simulink model "model_file_sim1"  (R2026b)
settings: Solver=FixedStepAuto  StopTime=stopTimeSimu  FixedStep=Ts
values from neighbouring files (symbols this model uses):
  Rc_alu = 11.0    (= 11)    [model.m]
  Rc_fan = 3.33    [model.m]
  Rc_fan1 = 3.33    [model.m]
  Rc_pet = 28.9    [model.m]
  Rc_pet1 = 28.9    [model.m]
  Rth_alu = 1.84 / 2    (= 0.92)    [model.m]
  Rth_alu2 = 1.84 / 2    (= 0.92)    [model.m]
  Rth_fan = 65.0 / 2    (= 32.5)    [model.m]
  Rth_fan2 = 65.0 / 2    (= 32.5)    [model.m]
  Rth_pet = 22.5 / 2    (= 11.25)    [model.m]
  Rth_pet2 = 22.5 / 2    (= 11.25)    [model.m]
  Rth_sen = 180.0    (= 180)    [model.m]
  Rv = 3.1    [model.m]
  Ts = 1    [R_from_logs.mat]    (also in estimate_R.m; kalman_manuel.m; kalman_simulink.m; model_file.m)
libraries: fl_lib x27, nesl_utility x4
settings Model: Creator=33683  LastModifiedBy=nael
settings DataIOCC: DSMLogging=off  ExternalInput=data_in  LoadExternalInput=on  ReturnWorkspaceOutputs=off  SaveOutput=off  SaveTime=off  SignalLogging=off
settings RTWCC: GPUComputeCapability=5.0
settings SimscapeCC: SimscapeUseEnergyAccounting=off

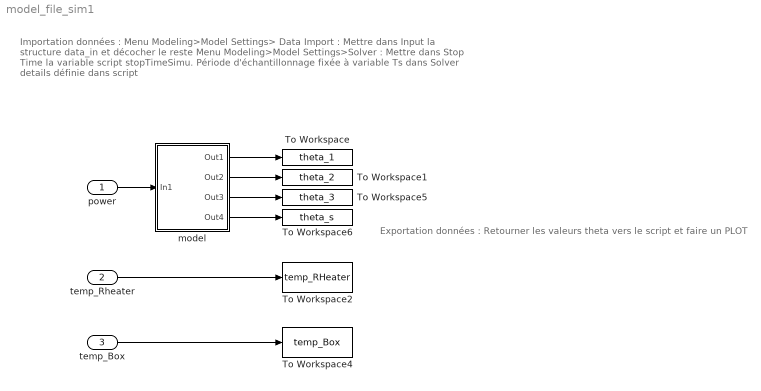
== system model_file_sim1 ==
  note: Importation données :
      | Menu Modeling>Model Settings> Data Import : Mettre dans Input la structure data_in et décocher le reste
      | Menu Modeling>Model Settings>Solver : Mettre dans Stop Time la variable script stopTimeSimu. Période d'échantillonnage fixée à variable Ts dans Solver details définie dans script
  note: Exportation données : Retourner les valeurs theta vers le script et faire un PLOT
  power : Inport
  temp_Rheater : Inport  Port=2
  temp_Box : Inport  Port=3
  To Workspace : ToWorkspace  VariableName=theta_1  SampleTime=Ts
  To Workspace1 : ToWorkspace  VariableName=theta_2  SampleTime=Ts
  To Workspace2 : ToWorkspace  VariableName=temp_RHeater  SampleTime=Ts
  To Workspace4 : ToWorkspace  VariableName=temp_Box  SampleTime=Ts
  To Workspace5 : ToWorkspace  VariableName=theta_3  SampleTime=Ts
  To Workspace6 : ToWorkspace  VariableName=theta_s  SampleTime=Ts
  model : Subsystem
  wires:
  temp_Rheater/1 -> To Workspace2/1
  temp_Box/1 -> To Workspace4/1
  power/1 -> model/1(In1)
  model/1(Out1) -> To Workspace/1
  model/2(Out2) -> To Workspace1/1
  model/3(Out3) -> To Workspace5/1
  model/4(Out4) -> To Workspace6/1

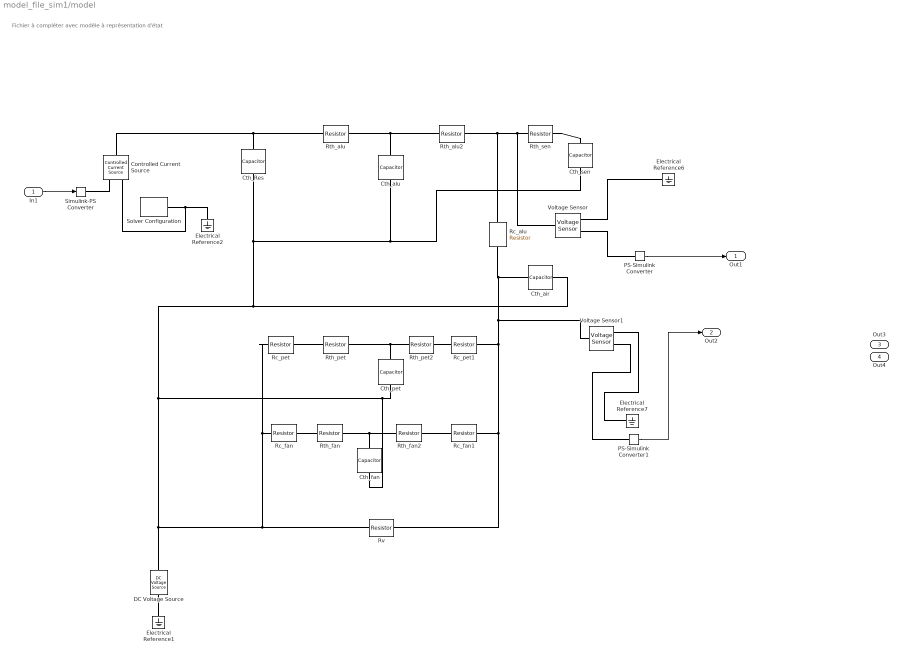
== system model_file_sim1/model ==
  note: Fichier à compléter avec modèle à représentation d'état
  In1 : Inport
  Controlled Current Source : fl_lib/Electrical/Electrical Sources/Controlled Current Source
  Cth_Res : fl_lib/Electrical/Electrical Elements/Capacitor  c=Cth_Res F  r=0 Ohm  g=0 1/Ohm  i_specify=off  i_priority=None  i=0 A  i_nominal_specify=off  i_nominal_value=1  i_nominal_unit=A  v_specify=off  v_priority=None  v=0 V  v_nominal_specify=off  v_nominal_value=1  v_nominal_unit=V  vc_specify=off  vc_priority=High  vc=0 V  vc_nominal_specify=off  vc_nominal_value=1  vc_nominal_unit=V
  Cth_air : fl_lib/Electrical/Electrical Elements/Capacitor  c=Cth_air F  r=0 Ohm  g=0 1/Ohm  i_specify=off  i_priority=None  i=0 A  i_nominal_specify=off  i_nominal_value=1  i_nominal_unit=A  v_specify=off  v_priority=None  v=0 V  v_nominal_specify=off  v_nominal_value=1  v_nominal_unit=V  vc_specify=off  vc_priority=High  vc=0 V  vc_nominal_specify=off  vc_nominal_value=1  vc_nominal_unit=V
  Cth_alu : fl_lib/Electrical/Electrical Elements/Capacitor  c=Cth_alu F  r=0 Ohm  g=0 1/Ohm  i_specify=off  i_priority=None  i=0 A  i_nominal_specify=off  i_nominal_value=1  i_nominal_unit=A  v_specify=off  v_priority=None  v=0 V  v_nominal_specify=off  v_nominal_value=1  v_nominal_unit=V  vc_specify=off  vc_priority=High  vc=0 V  vc_nominal_specify=off  vc_nominal_value=1  vc_nominal_unit=V
  Cth_fan : fl_lib/Electrical/Electrical Elements/Capacitor  c=Cth_fan F  r=0 Ohm  g=0 1/Ohm  i_specify=off  i_priority=None  i=0 A  i_nominal_specify=off  i_nominal_value=1  i_nominal_unit=A  v_specify=off  v_priority=None  v=0 V  v_nominal_specify=off  v_nominal_value=1  v_nominal_unit=V  vc_specify=off  vc_priority=High  vc=0 V  vc_nominal_specify=off  vc_nominal_value=1  vc_nominal_unit=V
  Cth_pet : fl_lib/Electrical/Electrical Elements/Capacitor  c=Cth_pet F  r=0 Ohm  g=0 1/Ohm  i_specify=off  i_priority=None  i=0 A  i_nominal_specify=off  i_nominal_value=1  i_nominal_unit=A  v_specify=off  v_priority=None  v=0 V  v_nominal_specify=off  v_nominal_value=1  v_nominal_unit=V  vc_specify=off  vc_priority=High  vc=0 V  vc_nominal_specify=off  vc_nominal_value=1  vc_nominal_unit=V
  Cth_sen : fl_lib/Electrical/Electrical Elements/Capacitor  c=Cth_sen F  r=0 Ohm  g=0 1/Ohm  i_specify=off  i_priority=None  i=0 A  i_nominal_specify=off  i_nominal_value=1  i_nominal_unit=A  v_specify=off  v_priority=None  v=0 V  v_nominal_specify=off  v_nominal_value=1  v_nominal_unit=V  vc_specify=off  vc_priority=High  vc=0 V  vc_nominal_specify=off  vc_nominal_value=1  vc_nominal_unit=V
  DC Voltage Source : fl_lib/Electrical/Electrical Sources/DC Voltage Source  v0=22 V
  Electrical Reference{1..2,6..7} (4 alike) : fl_lib/Electrical/Electrical Elements/Electrical Reference
  PS-Simulink Converter : nesl_utility/PS-Simulink Converter  PhysicalDomain=network_engine_domain  SubClassName=ps_output  LeftPortType=input  RightPortType=output  PseudoPeriodic=off  Frequencies=[]  VectorFormat=inherit  Unit=inherit  AffineConversion=off
  PS-Simulink Converter1 : nesl_utility/PS-Simulink Converter  PhysicalDomain=network_engine_domain  SubClassName=ps_output  LeftPortType=input  RightPortType=output  PseudoPeriodic=off  Frequencies=[]  VectorFormat=inherit  Unit=inherit  AffineConversion=off
  Rc_alu : fl_lib/Electrical/Electrical Elements/Resistor  R=Rc_alu Ohm  i_specify=off  i_priority=None  i=0 A  i_nominal_specify=off  i_nominal_value=1  i_nominal_unit=A  v_specify=off  v_priority=None  v=0 V  v_nominal_specify=off  v_nominal_value=1  v_nominal_unit=V
  Rc_fan : fl_lib/Electrical/Electrical Elements/Resistor  R=Rc_fan Ohm  i_specify=off  i_priority=None  i=0 A  i_nominal_specify=off  i_nominal_value=1  i_nominal_unit=A  v_specify=off  v_priority=None  v=0 V  v_nominal_specify=off  v_nominal_value=1  v_nominal_unit=V
  Rc_fan1 : fl_lib/Electrical/Electrical Elements/Resistor  R=Rc_fan1 Ohm  i_specify=off  i_priority=None  i=0 A  i_nominal_specify=off  i_nominal_value=1  i_nominal_unit=A  v_specify=off  v_priority=None  v=0 V  v_nominal_specify=off  v_nominal_value=1  v_nominal_unit=V
  Rc_pet : fl_lib/Electrical/Electrical Elements/Resistor  R=Rc_pet Ohm  i_specify=off  i_priority=None  i=0 A  i_nominal_specify=off  i_nominal_value=1  i_nominal_unit=A  v_specify=off  v_priority=None  v=0 V  v_nominal_specify=off  v_nominal_value=1  v_nominal_unit=V
  Rc_pet1 : fl_lib/Electrical/Electrical Elements/Resistor  R=Rc_pet1 Ohm  i_specify=off  i_priority=None  i=0 A  i_nominal_specify=off  i_nominal_value=1  i_nominal_unit=A  v_specify=off  v_priority=None  v=0 V  v_nominal_specify=off  v_nominal_value=1  v_nominal_unit=V
  Rth_alu : fl_lib/Electrical/Electrical Elements/Resistor  R=Rth_alu Ohm  i_specify=off  i_priority=None  i=0 A  i_nominal_specify=off  i_nominal_value=1  i_nominal_unit=A  v_specify=off  v_priority=None  v=0 V  v_nominal_specify=off  v_nominal_value=1  v_nominal_unit=V
  Rth_alu2 : fl_lib/Electrical/Electrical Elements/Resistor  R=Rth_alu2 Ohm  i_specify=off  i_priority=None  i=0 A  i_nominal_specify=off  i_nominal_value=1  i_nominal_unit=A  v_specify=off  v_priority=None  v=0 V  v_nominal_specify=off  v_nominal_value=1  v_nominal_unit=V
  Rth_fan : fl_lib/Electrical/Electrical Elements/Resistor  R=Rth_fan Ohm  i_specify=off  i_priority=None  i=0 A  i_nominal_specify=off  i_nominal_value=1  i_nominal_unit=A  v_specify=off  v_priority=None  v=0 V  v_nominal_specify=off  v_nominal_value=1  v_nominal_unit=V
  Rth_fan2 : fl_lib/Electrical/Electrical Elements/Resistor  R=Rth_fan2 Ohm  i_specify=off  i_priority=None  i=0 A  i_nominal_specify=off  i_nominal_value=1  i_nominal_unit=A  v_specify=off  v_priority=None  v=0 V  v_nominal_specify=off  v_nominal_value=1  v_nominal_unit=V
  Rth_pet : fl_lib/Electrical/Electrical Elements/Resistor  R=Rth_pet Ohm  i_specify=off  i_priority=None  i=0 A  i_nominal_specify=off  i_nominal_value=1  i_nominal_unit=A  v_specify=off  v_priority=None  v=0 V  v_nominal_specify=off  v_nominal_value=1  v_nominal_unit=V
  Rth_pet2 : fl_lib/Electrical/Electrical Elements/Resistor  R=Rth_pet2 Ohm  i_specify=off  i_priority=None  i=0 A  i_nominal_specify=off  i_nominal_value=1  i_nominal_unit=A  v_specify=off  v_priority=None  v=0 V  v_nominal_specify=off  v_nominal_value=1  v_nominal_unit=V
  Rth_sen : fl_lib/Electrical/Electrical Elements/Resistor  R=Rth_sen Ohm  i_specify=off  i_priority=None  i=0 A  i_nominal_specify=off  i_nominal_value=1  i_nominal_unit=A  v_specify=off  v_priority=None  v=0 V  v_nominal_specify=off  v_nominal_value=1  v_nominal_unit=V
  Rv : fl_lib/Electrical/Electrical Elements/Resistor  R=Rv Ohm  i_specify=off  i_priority=None  i=0 A  i_nominal_specify=off  i_nominal_value=1  i_nominal_unit=A  v_specify=off  v_priority=None  v=0 V  v_nominal_specify=off  v_nominal_value=1  v_nominal_unit=V
  Simulink-PS Converter : nesl_utility/Simulink-PS Converter  PhysicalDomain=network_engine_domain  SubClassName=ps_input  LeftPortType=input  RightPortType=output  PseudoPeriodic=off  Frequencies=[]  NoiseDistribution=none  NoiseParameters=[]  Unit=1  AffineConversion=off  FilteringAndDerivatives=provide  SimscapeFilterOrder=1  InputFilterTimeConstant=0.001  UdotUserProvided=0
  Solver Configuration : nesl_utility/Solver Configuration  PhysicalDomain=network_engine_domain  SubClassName=solver  LeftPortType=input  RightPortType=generic  Tones=[]  Harmonics=[]  SimulateNoise=off  Profile=off  UseLocalSampling=off  EnableSwitchedLinearOptims=on  FrequencyDomain=off  UseCCode=off  RelTol=0.001  AbsTol=0.001  MinStep=1e-09  ToWorkspace=off  RevertToSquareIcSolve=off  NumHomotopyIterations=100  PhasorMode=off  PhasorModeNumHarmonics=1  ConsistencySolver=NEWTON_XTOL_AFTER_FTOL  CanonicalOrdering=UNORDERED  OptimizeIntermediates=UNOPTIMIZED  MulticoreSolverChoice=BACKWARD_EULER  IndexReductionMethod=DerivativeReplacement  DoDC=off  ResidualTolerance=1e-09  ConsistencyTolSource=GLOBAL  ConsistencyAbsTol=0.001  ConsistencyRelTol=0.001  ConsistencyTolFactor=0.001  UseLocalSolver=off  LocalSolverChoice=NE_BACKWARD_EULER_ADVANCER  ResolveIndetEquations=on  FunctionEvalNumThread=1  LocalSolverSampleTime=0.001  DoFixedCost=off  MaxNonlinIter=3  MaxModeIter=2  ComputeImpulses=off  ImpulseIterations=2  LinearAlgebra=auto  LinearAlgebraNumThread=0  EquationFormulation=NE_TIME_EF  DelaysMemoryBudget=1024  AutomaticFiltering=on  FilteringTimeConstant=0.001  PartitionStorageMethod=AS_NEEDED  PartitionMemoryBudget=1024  PartitionMethod=BALANCED  MultibodyUseLocalSolver=off  MultibodyLocalSolverChoice=ODE1  MultibodyLocalSolverSampleTime=0.001
  Voltage Sensor : fl_lib/Electrical/Electrical Sensors/Voltage Sensor
  Voltage Sensor1 : fl_lib/Electrical/Electrical Sensors/Voltage Sensor
  Out1 : Outport
  Out2 : Outport  Port=2
  Out3 : Outport  Port=3
  Out4 : Outport  Port=4
  wires:
  PS-Simulink Converter1/1 -> Out2/1
  PS-Simulink Converter/1 -> Out1/1
  In1/1 -> Simulink-PS Converter/1
  connections:
  Cth_air/RConn1 -- Rc_fan/LConn1 -- Rc_pet/LConn1 -- Rv/LConn1 -- DC Voltage Source/LConn1 -- Cth_pet/RConn1 -- Cth_fan/RConn1 -- Cth_sen/RConn1 -- Cth_alu/RConn1 -- Cth_Res/RConn1
  Rth_fan/RConn1 -- Rth_fan2/LConn1 -- Cth_fan/LConn1
  Rth_sen/LConn1 -- Voltage Sensor/LConn1 -- Rc_alu/LConn1 -- Rth_alu2/RConn1
  Rth_alu/RConn1 -- Cth_alu/LConn1 -- Rth_alu2/LConn1
  Rth_pet2/LConn1 -- Rth_pet/RConn1 -- Cth_pet/LConn1
  Rth_pet/LConn1 -- Rc_pet/RConn1
  Electrical Reference7/LConn1 -- Voltage Sensor1/RConn2
  Rc_pet1/LConn1 -- Rth_pet2/RConn1
  Voltage Sensor1/RConn1 -- PS-Simulink Converter1/LConn1
  DC Voltage Source/RConn1 -- Electrical Reference1/LConn1
  Rc_fan1/LConn1 -- Rth_fan2/RConn1
  Rth_sen/RConn1 -- Cth_sen/LConn1
  Voltage Sensor/RConn2 -- Electrical Reference6/LConn1
  Voltage Sensor/RConn1 -- PS-Simulink Converter/LConn1
  Rth_fan/LConn1 -- Rc_fan/RConn1
  Solver Configuration/RConn1 -- Electrical Reference2/LConn1 -- Controlled Current Source/RConn2
  Simulink-PS Converter/RConn1 -- Controlled Current Source/RConn1
  Rth_alu/LConn1 -- Controlled Current Source/LConn1 -- Cth_Res/LConn1
  Rv/RConn1 -- Rc_fan1/RConn1 -- Rc_pet1/RConn1 -- Voltage Sensor1/LConn1 -- Rc_alu/RConn1 -- Cth_air/LConn1
